simulink model "advanced_bms_aco_ekf"  (R2024b)
settings: Solver=FixedStepDiscrete  StartTime=0.0  StopTime=BMS_StopTime  FixedStep=1  RelTol=1e-3
InitFcn:
  | bms_setup('synthetic')
values from neighbouring files (symbols this model uses):
  BMS_Q : value not decoded    [bms_data.sldd]
  BMS_R = 0.001474701    [bms_data.sldd]
undefined symbols (not defined in the file or in its folder): BMS_FaultMode, BMS_Seed, BMS_SOC0, BMS_SOC_Guess
settings Model: DataDictionary=bms_data.sldd  Creator=sande  LastModifiedBy=sande
settings DataIOCC: SaveOutput=off
settings DebuggingCC: SignalInfNanChecking=error  AlgebraicLoopMsg=error  ArtificialAlgebraicLoopMsg=error  UnconnectedInputMsg=error  UnconnectedOutputMsg=error  UnconnectedLineMsg=error  BusObjectLabelMismatch=error  StrictBusMsg=ErrorOnBusTreatedAsVector
settings HardwareCC: ProdBitPerPointer=32  ProdBitPerSizeT=32  ProdBitPerPtrDiffT=32  ProdLargestAtomicInteger=Long  ProdLargestAtomicFloat=Double  ProdWordSize=32  ProdHWDeviceType=ARM Compatible->ARM Cortex

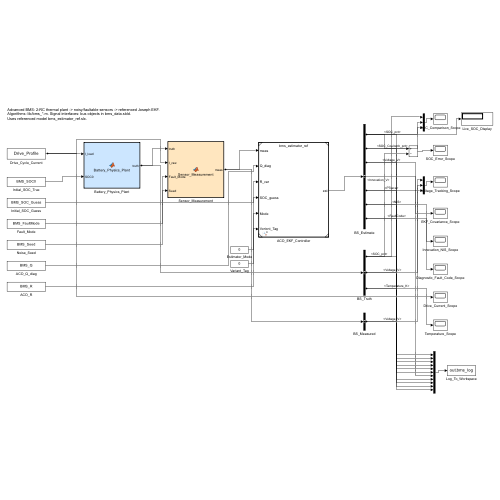
[thumbnail: Simulink's stored preview of the top-level diagram]
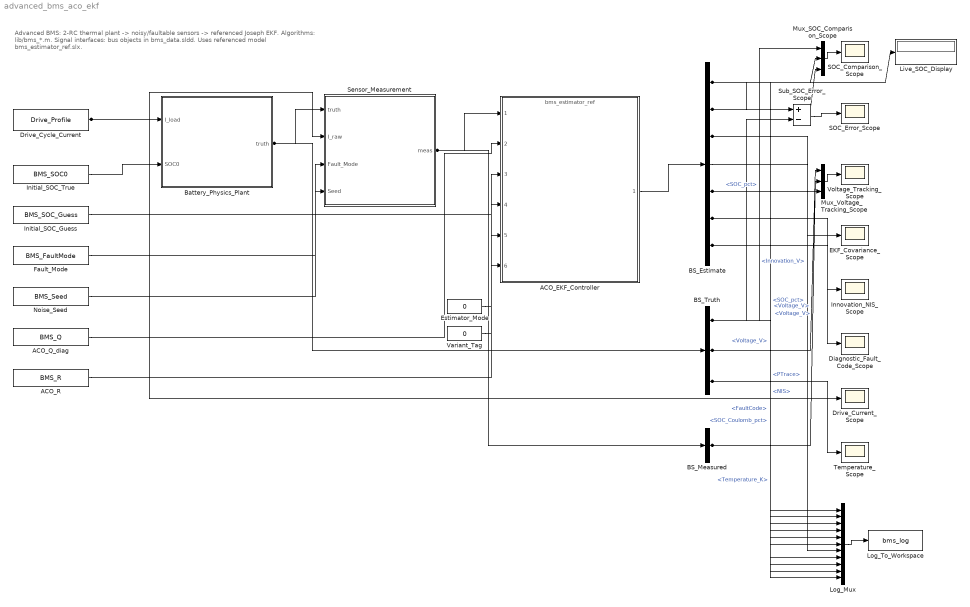
== system advanced_bms_aco_ekf ==
  note: Advanced BMS: 2-RC thermal plant -> noisy/faultable sensors -> referenced Joseph EKF.
      | Algorithms: lib/bms_*.m. Signal interfaces: bus objects in bms_data.sldd.
      | Uses referenced model bms_estimator_ref.slx.
  ACO_EKF_Controller : ModelReference  ModelNameDialog=bms_estimator_ref  SimulationMode=Normal  ModelReferenceVersion=1.2
  ACO_Q_diag : Constant  Value=BMS_Q  SampleTime=-1
  ACO_R : Constant  Value=BMS_R  SampleTime=-1
  BS_Estimate : BusSelector  OutputSignals=SOC_pct,SOC_Coulomb_pct,Voltage_V,Innovation_V,PTrace,NIS,FaultCode
  BS_Measured : BusSelector  OutputSignals=Voltage_V
  BS_Truth : BusSelector  OutputSignals=SOC_pct,Voltage_V,Temperature_K
  Battery_Physics_Plant : MATLAB Function  TreatAsAtomicUnit=on
  Diagnostic_Fault_Code_Scope : Scope
      settings: Description=1 V range | 2 T range | 4 I range | 8 innovation rejected | 16 filter inconsistent
  Drive_Current_Scope : Scope
      settings: Description=Current [A]
  Drive_Cycle_Current : FromWorkspace  VariableName=Drive_Profile  SampleTime=1  Interpolate=off  OutputAfterFinalValue=Holding final value
  EKF_Covariance_Scope : Scope
      settings: Description=trace(P)
  Estimator_Mode : Constant  Value=0  SampleTime=-1
  Fault_Mode : Constant  Value=BMS_FaultMode  SampleTime=-1
  Initial_SOC_Guess : Constant  Value=BMS_SOC_Guess  SampleTime=-1
  Initial_SOC_True : Constant  Value=BMS_SOC0  SampleTime=-1
  Innovation_NIS_Scope : Scope
      settings: Description=Normalised innovation squared (expect ~1)
  Live_SOC_Display : Display
  Log_Mux : Mux  Inputs=11
  Log_To_Workspace : ToWorkspace  VariableName=bms_log  SampleTime=-1
  Mux_SOC_Comparison_Scope : Mux  Inputs=3
  Mux_Voltage_Tracking_Scope : Mux  Inputs=3
  Noise_Seed : Constant  Value=BMS_Seed  SampleTime=-1
  SOC_Comparison_Scope : Scope
      settings: Description=True SOC | EKF SOC | Coulomb counting
  SOC_Error_Scope : Scope
      settings: Description=EKF - True [%]
  Sensor_Measurement : MATLAB Function  TreatAsAtomicUnit=on
  Sub_SOC_Error_Scope : Sum  Inputs=+-
  Temperature_Scope : Scope
      settings: Description=Cell temperature [K]
  Variant_Tag : Constant  Value=0  SampleTime=-1
  Voltage_Tracking_Scope : Scope
      settings: Description=True V | Measured V | EKF predicted V
  wires:
  Drive_Cycle_Current/1 -> Battery_Physics_Plant/1(I_load), Sensor_Measurement/2(I_raw), Drive_Current_Scope/1
  Initial_SOC_True/1 -> Battery_Physics_Plant/2(SOC0)
  Battery_Physics_Plant/1(truth) -> Sensor_Measurement/1(truth), BS_Truth/1
  Fault_Mode/1 -> Sensor_Measurement/3(Fault_Mode)
  Noise_Seed/1 -> Sensor_Measurement/4(Seed)
  Sensor_Measurement/1(meas) -> ACO_EKF_Controller/1, BS_Measured/1
  ACO_Q_diag/1 -> ACO_EKF_Controller/2
  ACO_R/1 -> ACO_EKF_Controller/3
  Initial_SOC_Guess/1 -> ACO_EKF_Controller/4
  Estimator_Mode/1 -> ACO_EKF_Controller/5
  Variant_Tag/1 -> ACO_EKF_Controller/6
  ACO_EKF_Controller/1 -> BS_Estimate/1
  BS_Truth/1 -> Mux_SOC_Comparison_Scope/1, Sub_SOC_Error_Scope/2, Log_Mux/1  "<SOC_pct>"
  BS_Estimate/1 -> Mux_SOC_Comparison_Scope/2, Sub_SOC_Error_Scope/1, Live_SOC_Display/1, Log_Mux/2  "<SOC_pct>"
  BS_Estimate/2 -> Mux_SOC_Comparison_Scope/3, Log_Mux/3  "<SOC_Coulomb_pct>"
  Mux_SOC_Comparison_Scope/1 -> SOC_Comparison_Scope/1
  Sub_SOC_Error_Scope/1 -> SOC_Error_Scope/1
  BS_Truth/2 -> Mux_Voltage_Tracking_Scope/1, Log_Mux/4  "<Voltage_V>"
  BS_Measured/1 -> Mux_Voltage_Tracking_Scope/2, Log_Mux/5  "<Voltage_V>"
  BS_Estimate/3 -> Mux_Voltage_Tracking_Scope/3, Log_Mux/6  "<Voltage_V>"
  Mux_Voltage_Tracking_Scope/1 -> Voltage_Tracking_Scope/1
  BS_Estimate/5 -> EKF_Covariance_Scope/1, Log_Mux/8  "<PTrace>"
  BS_Estimate/6 -> Innovation_NIS_Scope/1, Log_Mux/9  "<NIS>"
  BS_Estimate/7 -> Diagnostic_Fault_Code_Scope/1, Log_Mux/10  "<FaultCode>"
  BS_Truth/3 -> Temperature_Scope/1, Log_Mux/11  "<Temperature_K>"
  BS_Estimate/4 -> Log_Mux/7  "<Innovation_V>"
  Log_Mux/1 -> Log_To_Workspace/1

== matlab function advanced_bms_aco_ekf/Sensor_Measurement ==
  data: truth input Bus: BMS_PlantTruth; meas output Bus: BMS_Measurement; I_raw input; Fault_Mode input; Seed input
function meas = Sensor_Measurement(truth, I_raw, Fault_Mode, Seed)
%#codegen
% Noisy 12-bit-class sensors with injectable faults. Algorithm: lib/bms_sensor_step.m (seeded, reproducible)
% Input: bus BMS_PlantTruth. Output: bus BMS_Measurement
P = coder.const(bms_params('synthetic'));
persistent ss k;
if isempty(ss)
    ss = bms_seed(Seed);  k = 0.0;
end
k = k + 1.0;
[Vm, Im, Tm, ss] = bms_sensor_step(truth.Voltage_V, I_raw, truth.Temperature_K, k, ss, P, Fault_Mode);
meas.Voltage_V = Vm;
meas.Current_A = Im;
meas.Temperature_K = Tm;

== matlab function advanced_bms_aco_ekf/Battery_Physics_Plant ==
  data: I_load input; truth output Bus: BMS_PlantTruth; SOC0 input
function truth = Battery_Physics_Plant(I_load, SOC0)
%#codegen
% 2-RC Arrhenius cell with capacity/resistance mismatch (see bms_params). Algorithm: lib/bms_plant_step.m
% Output: bus BMS_PlantTruth
P = coder.const(bms_params('synthetic'));
persistent x k;
if isempty(x)
    x = [SOC0; 0.0; 0.0];  k = 0.0;
end
k = k + 1.0;
T = bms_temp_profile(k);
[x, Vt] = bms_plant_step(x, I_load, T, P);
truth.SOC_pct = 100.0 * x(1);
truth.Voltage_V = Vt;
truth.Temperature_K = T;
